simulink model "tractor_mu2018"  (R2018a)
settings: Solver=FixedStepDiscrete  StartTime=0.0  StopTime=30  FixedStep=0.001  RelTol=1e-3
model workspace (MAT data in the model file):
  MCOS : class17 (value not decoded)
undefined symbols (not defined in the file): A, a, B, b, C, D, DiscIntNeverNeededParam, Iz, K, k1, K1, k2, K2, L1, L2, m, magnitude, Phi, Sample_time, Steer_Ratio
libraries: simulink x39, Solver_SF x1, dsparch4 x1
(part 4 of 5)

== matlab function tractor_mu2018/四轮转矩分配/MATLAB Function ==
  data: Mz input; Tfl output; Tfr output; Trl output; Trr output; T0 input; derta input; k input; mode input
function [Tfl,Tfr,Trl,Trr] = fcn(Mz,T0,derta,k,mode)
rf = single(0.834);
rr = single(0.94);
df = single(2.39);
dr = single(2.33);
a = single(2.043);

Trr = single(0);
Trl = single(0);
Tfl = single(0);
Tfr = single(0);


% 强制将输入 Mz 类型设为 single，避免隐式转换
Mz = single(Mz);
T0 = single(T0);
derta = single(derta);
mode = single(mode);

% if mode == 5 || mode == 6
%     k = single(3/7); 
% elseif mode == 1 || mode == 3 
%     k = min(k,1);
%     k = max(k,0.3);
% end

A = T0 / (k + single(1));
B = (Mz - a*sin(derta)*k*A/rf) / (df*cos(derta)*k*rr + dr*rf) * (2*rf*rr);
Trr = (A + B) / single(2);
Trl = (A - B) / single(2);
Tfl = k * Trl;
Tfr = k * Trr;

== matlab function tractor_mu2018/Dugoff轮胎模型/pac2002/rl_dugoff ==
  data: Fz input; Fx0 output; u input; lamda input; alpha input; Fy0 output; Fx output; Fy output
function [Fx0,Fy0,Fx,Fy] = tire(Fz,u,lamda,alpha)
cx = -20;
cy = -20;
L = (1-lamda)/(2*sqrt(cx^2*lamda^2+cy^2*(tan(alpha))^2));
if L<1
    fL = L*(2-L);
else
    fL = 1;
end
Fx0 = Fz*cx*lamda*fL/(1-lamda);
Fy0 = Fz*cy*tan(alpha)*fL/(1-lamda);
Fx = u*Fx0;
Fy = u*Fy0;

== matlab function tractor_mu2018/Dugoff轮胎模型/pac2002/rr_dugoff ==
  data: Fz input; Fx0 output; u input; lamda input; alpha input; Fy0 output; Fx output; Fy output
function [Fx0,Fy0,Fx,Fy] = tire(Fz,u,lamda,alpha)
cx = -20;
cy = -20;
L = (1-lamda)/(2*sqrt((cx^2)*(lamda^2)+(cy^2)*((tan(alpha))^2)));
if L<1
    fL = L*(2-L);
else
    fL = 1;
end
Fx0 = Fz*cx*lamda*fL/(1-lamda);
Fy0 = Fz*cy*tan(alpha)*fL/(1-lamda);
Fx = u*Fx0;
Fy = u*Fy0;

== matlab function tractor_mu2018/质心侧偏角估计/define_Kalman ==
  data: u input; A output; B output; C output; D output; a11 output; a12 output; a21 output single; a22 output; c11 output; c12 output
function [A, B, C, D,a11,a12,a21,a22,c11,c12] = fcn(u)
m = 18530;%质量
Iz = 67536;%绕Z轴的转动惯量
a = 2.043;%前轴距
b=1.362;%后轴距
% k1 = -1360400;%前侧偏刚度
% k2 = -1611200;%后侧偏刚度
k1 = -304828*2;%前侧偏刚度
k2 = -417040*2;%后侧偏刚度
t = 0.001;%仿真步长
Sample_time = 0.001;


a11 = (k1+k2)*t/(m*u)+1;
a12 = ((a*k1-b*k2)/(m*u^2)-1)*t;
a21 = single((a*k1-b*k2)*t/Iz);
a22 = (a^2*k1+b^2*k2)*t/(Iz*u)+1;
b11  =-k1*t/(m*u);
b21 = -a*k1*t/Iz;
c11 = (k1+k2)/m;
c12 = (a*k1-b*k2)/(m*u);
c21 = 0;
c22 = 1;
d11 = -k1/m;
d21 = 0;

%% A B C D 为kalman滤波器中各个矩阵

A = [a11 a12;a21 a22];
B = [b11;b21];
C = [c11 c12;c21 c22];
D = [d11;d21];

== matlab function tractor_mu2018/驱动防滑模块/MATLAB Function ==
  data: sp1 input; vfl output; sp2 input; vfr output
function [vfl,vfr] = fcn(sp1,sp2)
r1 = 0.834;

if sp1>=0
    vfl = max(0.001,sp1*2*pi*r1/60); %m/s
else
    vfl = min(-0.001,sp1*2*pi*r1/60); %m/s
end

if sp2 >= 0
    vfr = max(0.001,sp2*2*pi*r1/60);
else
    vfr = min(0.001,sp2*2*pi*r1/60);
end

== matlab function tractor_mu2018/驱动防滑模块/MATLAB Function1 ==
  data: sp3 input; vrl output; sp4 input; vrr output
function [vrl,vrr] = fcn(sp3,sp4)
r2 = 0.94;

if sp3 >= 0
    vrl = max(0.001,sp3*2*pi*r2/60);
else
    vrl = min(0.001,sp3*2*pi*r2/60);
end

if sp4 >=0
    vrr = max(0.001,sp4*2*pi*r2/60);
else
    vrr = min(0.001,sp4*2*pi*r2/60);
end

== stateflow chart tractor_mu2018/驱动防滑模块/转矩协调控制 ==
  state coordinate
    (default) -> (junction 7)
    (junction 7) -> (junction 9) [order 1] : [dT1 ~= 0]
    (junction 9) -> (junction 11) [order 1] : [dT2 ~= 0]
    (junction 11) -> (junction 14) [order 1] : [abs(dT1)>=abs(dT2)]{dTfr=dT1;dTfl=dT1;}
    (junction 14) -> (junction 16)
    (junction 7) -> (junction 21) [order 2] : {dTfr=dT2;
        | dTfl=dT2}
    (junction 9) -> (junction 19) [order 2] : {dTfr=dT1;
        | dTfl=dT1;}
    (junction 11) -> (junction 16) [order 2] : {dTfr=dT2;dTfl=dT2;}
    (junction 19) -> (junction 21)
    (junction 16) -> (junction 19)
    (junction 21) -> (junction 111)
    (junction 111) -> (junction 106) [order 2] : {dTrr=dT4;
        | dTrl=dT4}
    (junction 111) -> (junction 118) [order 1] : [dT3 ~= 0]
    (junction 118) -> (junction 107) [order 1] : [dT4 ~= 0]
    (junction 107) -> (junction 110) [order 1] : [abs(dT3)>=abs(dT4)]{dTrr=dT3;dTrl=dT3;}
    (junction 110) -> (junction 114)
    (junction 115) -> (junction 106)
    (junction 118) -> (junction 115) [order 2] : {dTrr=dT3;
        | dTrl=dT3;}
    (junction 107) -> (junction 114) [order 2] : {dTrr=dT4;dTrl=dT4;}
    (junction 114) -> (junction 115)
  state no_coordinate
    du:
    dTfl=dT1;
    dTfr=dT2;
    dTrl=dT3;
    dTrr=dT4;
  (default) -> (junction 123)
  (junction 123) -> (junction 126) [order 2]
  (junction 123) -> no_coordinate [order 1] : [v<10]
  (junction 126) -> coordinate
  no_coordinate -> coordinate : [v>=10]
  coordinate -> no_coordinate [order 1] : [v<10]
  coordinate -> coordinate [order 2] : [v>=10]
  data: v input; dT1 input; dT2 input; dT3 input; dT4 input; dTfl output; dTfr output; dTrl output; dTrr output

== matlab function tractor_mu2018/四轮转矩分配/MATLAB Function1 ==
  data: X_current input; U_optimal output; Fx input; Mz input; Fz_all input; mu input; last_U_in input
function U_optimal = mpc_torque_allocation_fcn(X_current, Fx, Mz, Fz_all, mu, last_U_in)
% 基于MPC的四轮驱动车辆扭矩分配。
% 本函数在每个计算步中构建并求解一个二次规划(QP)问题。

%#codegen

% -------------------------------------------------------------------------
% 1. 定义持久化变量和参数
% -------------------------------------------------------------------------
% persistent 关键字定义的变量只在第一次调用函数时初始化，之后会保持它们的值。
persistent vehicle_params mpc_params last_U

if isempty(vehicle_params)
    % --- 车辆参数 ---
    % !! 请根据您的拖拉机模型修改以下参数 !!
    vehicle_params.m = 18530;   % 质量 (kg)
    vehicle_params.Iz = 67536;  % 绕Z轴的转动惯量 (kg*m^2)
    vehicle_params.lf = 2.043;   % 质心到前轴的距离 (m)
    vehicle_params.lr = 1.362;   % 质心到后轴的距离 (m)
    vehicle_params.wf = 2.39;    % 前轮距 (m)
    vehicle_params.wr = 2.33;    % 后轮距 (m)

    % --- MPC 参数 ---
    mpc_params.Ts = 0.001;      % 采样时间 (s)，必须与Simulink的采样时间一致
    mpc_params.Np = 20;        % 预测时域 (Prediction Horizon)
    mpc_params.Nc = 10;         % 控制时域 (Control Horizon)
    
    % --- MPC 权重 ---
    % 对控制输入变化率 (delta U) 的惩罚矩阵R的对角线元素
    mpc_params.R_diag = ones(8, 1) * 0.01; 
    mpc_params.w_ax = 1.0;      % 纵向加速度权重
    mpc_params.w_ay = 1;      % 横向加速度权重
    
    % --- 轮胎附着多边形 ---
    % 使用一个八边形来线性化近似摩擦圆约束
    num_sides = 8;
    angles = (0:num_sides-1)' * (2*pi/num_sides);
    mpc_params.friction_polygon = [cos(angles), sin(angles)]; % [cos, sin] 列
    
    % 初始化上一次的控制输入
    last_U = zeros(8, 1);
end

% 从输入端口更新last_U，以保证时间步之间的一致性
if any(size(last_U_in) ~= size(last_U))
   last_U = zeros(8,1); % 如果是第一次运行或尺寸不匹配，则进行初始化
else
   last_U = last_U_in;
end


% -------------------------------------------------------------------------
% 2. 获取参数
% -------------------------------------------------------------------------
% 车辆参数
m = vehicle_params.m;
Iz = vehicle_params.Iz;
lf = vehicle_params.lf;
lr = vehicle_params.lr;
wf = vehicle_params.wf;
wr = vehicle_params.wr;
bf = wf / 2; % 半轮距
br = wr / 2;

% MPC参数
Ts = mpc_params.Ts;
Np = mpc_params.Np;
Nc = mpc_params.Nc;
R = diag(mpc_params.R_diag);

% 解析输入信号
u_k = X_current(1); % 当前的纵向车速 (m/s)
v_k = X_current(2); % 当前的横向车速 (m/s)
r_k = X_current(3); % 当前横摆角速度 (rad/s)

% -------------------------------------------------------------------------
% 3. 定义状态空间矩阵 
% -------------------------------------------------------------------------
% 连续时间的状态矩阵 A_c，它依赖于当前车速 u_k
A_c = [0, 0, 0;
       0, 0, u_k;
       0, 0, 0];

% 连续时间的输入矩阵 B_c  横摆方向逆时针为正;横向向左为正
B_c = [1/m,   0,   1/m,   0,   1/m,   0,   1/m,   0;
       0,   1/m,   0,   1/m,   0,   1/m,   0,   1/m;
       -bf/Iz, lf/Iz, bf/Iz, lf/Iz, -br/Iz, -lr/Iz, br/Iz, -lr/Iz];

% 使用前向欧拉法进行离散化
Ad = eye(3) + A_c * Ts;
Bd = B_c * Ts;

% -------------------------------------------------------------------------
% 4. 构建二次规划(QP)问题 
%    目标: min 0.5 * dU' * H * dU + f' * dU
% -------------------------------------------------------------------------
% 新代价函数: J = sum( (ax^2+ay^2) + dU'*R*dU )

% ---- 4.1 定义权重和矩阵 ----
% 从参数区获取加速度权重
w_ax = mpc_params.w_ax;
w_ay = mpc_params.w_ay;
Q_accel = diag([w_ax^2, w_ay^2]); % 单步的加速度权重矩阵

% 构建整个控制时域的权重矩阵
Q_bar = kron(eye(Nc), Q_accel);  % 加速度项的权重矩阵
R_bar = kron(eye(Nc), R);      % 控制增量项的权重矩阵

% ---- 4.2 将加速度表示为dU的函数 ----
% 定义一个矩阵，从控制向量U中提取与加速度相关的力
C_u = [1/m, 0, 1/m, 0, 1/m, 0, 1/m, 0;
       0, 1/m, 0, 1/m, 0, 1/m, 0, 1/m];
C_u_bar = kron(eye(Nc), C_u);

% 计算由当前状态(u_k, v_k, r_k)引起的加速度偏移量
% (在线性化过程中被视为常数)
d_accel_k = [-v_k * r_k; 2 * u_k * r_k];
d_accel_bar = repmat(d_accel_k, Nc, 1);

% ---- 4.3 构建QP矩阵 H 和 f ----
% 回忆: U_vec = M_sum * dU_vec + U_last_vec
% 预测的加速度 Accel_vec = C_u_bar * U_vec + d_accel_bar
%                        = C_u_bar * (M_sum * dU_vec + U_last_vec) + d_accel_bar
%                        = (C_u_bar * M_sum) * dU_vec + (C_u_bar * U_last_vec + d_accel_bar)
%
% 令 S = C_u_bar * M_sum
% 令 E = C_u_bar * U_last_vec + d_accel_bar
% 则 Accel_vec = S * dU_vec + E
%
% 加速度部分的代价 J_accel = (S*dU+E)' * Q_bar * (S*dU+E)
% 展开后与QP标准型对比，可以推导出H和f的构成

% 预先计算一个将 dU_vec 映射到 U_vec 的矩阵
% U_vec = M_sum * dU_vec + U_last_vec
M_sum = kron(tril(ones(Nc, Nc)), eye(8));
U_last_vec = repmat(last_U, Nc, 1);

S = C_u_bar * M_sum;
E = C_u_bar * U_last_vec + d_accel_bar;

% 构建 H 矩阵
H = 2 * (S' * Q_bar * S + R_bar);

% 构建 f 向量
f = 2 * (S' * Q_bar * E);

% ---- 4.2 构建约束矩阵 ----
% 优化变量是dU。所有约束都必须是关于dU的线性形式: A*dU <= b 或 Aeq*dU = beq
% 未来的控制量 U_k+i 与 增量 dU 的关系: U_k+i = U_{k-1} + dU_k + ... + dU_k+i



% --- 4.2.1 等式约束: Aeq * dU_vec = beq ---
% 在所有 Nc 控制步内，都满足 Fx_total = Fx_ref 和 Mz_total = Mz_ref
C_fx = [1, 0, 1, 0, 1, 0, 1, 0];
C_mz = [-bf, lf, bf, lf, -br, -lr, br, -lr]; % 注意: 此处未除以Iz，因为约束是针对力矩本身

Aeq_block = [C_fx; C_mz]; % (维度: 2 x 8)
Aeq = kron(eye(Nc), Aeq_block); % (维度: 2*Nc x 8*Nc)
Aeq = Aeq * M_sum;

% 构建等式约束右侧的beq向量
beq_fx = ones(Nc, 1) * Fx;
beq_mz = ones(Nc, 1) * Mz;
beq_block = [beq_fx'; beq_mz']; % (维度: 2 x Nc)
beq = beq_block(:); % (维度: 2*Nc x 1)
% 别忘了减去上个时刻控制量的影响
beq = beq - kron(eye(Nc), Aeq_block) * U_last_vec;

% --- 4.2.2 不等式约束: Aineq * dU_vec <= bineq ---
% 对所有4个轮胎、在所有Nc控制步内的轮胎附着多边形约束
% poly_sides = mpc_params.friction_polygon;
% num_sides = size(poly_sides, 1);
% num_tires = 4;
% 
% Aineq_block = zeros(num_sides * num_tires, 8);
% for i = 1:num_tires % 遍历: 左前, 右前, 左后, 右后
%     % 找到这个轮胎对应的Fx和Fy列的索引
%     idx_fx = 2*i - 1;
%     idx_fy = 2*i;
%     
%     % 获取这个轮胎对应约束的行索引范围
%     row_start = (i-1)*num_sides + 1;
%     row_end = i*num_sides;
%     
%     % 填充多边形约束系数
%     Aineq_block(row_start:row_end, idx_fx) = poly_sides(:, 1); % cos(theta)
%     Aineq_block(row_start:row_end, idx_fy) = poly_sides(:, 2); % sin(theta)
% end
% 
% Aineq = kron(eye(Nc), Aineq_block); % (维度: num_sides*num_tires*Nc x 8*Nc)
% Aineq = Aineq * M_sum;
% 
% % 构建不等式约束右侧的bineq向量
% mu_vec = ones(4,1) * mu; % 暂时假设所有轮胎的附着系数 mu 相同
% Fz_mu_vec = Fz_all .* mu_vec; % 计算每个轮胎的最大附着力
% bineq_block = repelem(Fz_mu_vec, num_sides, 1); % repelem for R2017a+, for older use kron
% bineq = repmat(bineq_block, Nc, 1);
% % 同样，减去上个时刻控制量的影响
% bineq = bineq - kron(eye(Nc), Aineq_block) * U_last_vec;

% -------------------------------------------------------------------------
% 5. 求解QP问题
% -------------------------------------------------------------------------
% 设置 quadprog 求解器选项
U_optimal = zeros(8,1);
options = optimoptions('quadprog', 'Display', 'none', 'Algorithm', 'active-set');

% 为求解器创建一个全零的初始猜测点 x0
% 它的维度必须与优化变量dU_vec一致 (8*Nc x 1)
x0 = zeros(8 * Nc, 1);

% --- 【新增代码】构建下界(lb)向量以保证驱动轮Fx >= 0 ---
% lb是直接作用于优化变量dU_vec的

% 首先，为单个时间步的dU创建一个下界向量
lb_step = -inf(8, 1);

% 假设所有4个轮子都只作为驱动轮，不能为负
% Fx的索引是 1, 3, 5, 7
drive_idx = [1, 3, 5, 7]; 
% Fx的增量的下界是上一时刻Fx的负值，以保证 Fx_k = Fx_{k-1} + dFx_k >= 0
lb_step(drive_idx) = -last_U(drive_idx);

% 然后，将单步的下界向量复制Nc次，以覆盖整个控制时域
lb = repmat(lb_step, Nc, 1);

% 【修改代码】调用求解器，将lb作为第7个参数传入
% [dU_vec_sol, ~, exitflag] = quadprog(H, f, Aineq, bineq, Aeq, beq, lb, [], x0, options);
[dU_vec_sol, ~, exitflag] = quadprog(H, f, [], [], Aeq, beq, lb, [], x0, options);
% -------------------------------------------------------------------------
% 6. 处理求解结果
% -------------------------------------------------------------------------
if exitflag == 1 % 返回1代表求解成功
    % 提取第一个控制增量 (Receding Horizon Control)
    dU_optimal = dU_vec_sol(1:8);
    % 计算当前时刻的最终控制输入
    U_optimal = last_U + dU_optimal;
else
    % 如果求解失败, 保持上一次的控制输入不变 (作为一种安全备用策略)
    U_optimal = last_U;
end

% 无需在此更新 last_U, 因为它会作为输出连接到Unit Delay模块，
% 并在下个采样时刻通过输入端口 last_U_in 传回。

end

== matlab function tractor_mu2018/Subsystem/MATLAB Function ==
  data: Fd input; P_qianyin input; y output; P_qudong input; v input
function y = fcn(Fd,P_qianyin,P_qudong,v)

if Fd > 0 && v > 0.5/3.6
    y = P_qianyin/P_qudong;
else
    y = 0;
end
if P_qudong < 2000
    y = 0;
end

== matlab function tractor_mu2018/四轮转矩分配/MATLAB Function2 ==
  data: F input; Tfl output; derta input; Tfr output; Trl output; Trr output; dwfl input; dwfr input; dwrl input; dwrr input
function [Tfl,Tfr,Trl,Trr] = fcn(F,derta,dwfl,dwfr,dwrl,dwrr)
% 向左为正
rf = 0.834;
rr = 0.94;
If = 110.64; % kg*m^2
Ir = 356.42;

Ffl = F(1)*cos(derta) + F(2)*sin(derta);
Tfl = Ffl*rf + If*dwfl;
Ffr = F(3)*cos(derta) + F(4)*sin(derta);
Tfr = Ffr*rf + If*dwfr;
Frl = F(5);
Trl = Frl*rr + Ir*dwrl;
Frr = F(7);
Trr = Frr*rr + Ir*dwrr;

== matlab function tractor_mu2018/驱动防滑模块/MATLAB Function2 ==
  data: v input; dTfl output; dT1 input; dT2 input; dT3 input; dT4 input; dTfr output; dTrl output; dTrr output
function [dTfl,dTfr,dTrl,dTrr] = fcn(v,dT1,dT2,dT3,dT4)

v = v*3.6;

if v < 1.5
    dTfl = 0;
    dTfr = 0;
    dTrl = 0;
    dTrr = 0;
end

if v < 10
    dTfl = dT1;
    dTfr = dT2;
    dTrl = dT3;
    dTrr = dT4;
else 
    if abs(dT1) > abs(dT2)
        dTfl = dT1;
        dTfr = dT1;
    else
        dTfl = dT2;
        dTfr = dT2;
    end
    if abs(dT3) > abs(dT4)
        dTrl = dT3;
        dTrr = dT3;
    else
        dTrl = dT4;
        dTrr = dT4;
    end
end

== stateflow chart tractor_mu2018/车轮腾空判断/FL ==
  state suspected
    airborne_flag = 0; confidence = 0.5;
  state grounded
    airborne_flag = 0; confidence = 0;
  state airborne
    airborne_flag = 1; confidence = 1;
  grounded -> suspected : [ (lamda > 0) && (Tload_hat < 50) && (domega > 0) && (abs(az)) > 2]
  suspected -> airborne : [after(0.02, sec)]
  (default) -> grounded
  airborne -> grounded : [(lamda < 0.02) && (Tload_hat > 100) && abs(az) < 1 && after(0.05,sec)]
  data: lamda input; Tload_hat input; az input; domega input; airborne_flag output; confidence output

== stateflow chart tractor_mu2018/车轮腾空判断/FR ==
  state suspected
    airborne_flag = 0; confidence = 0.5;
  state grounded
    airborne_flag = 0; confidence = 0;
  state airborne
    airborne_flag = 1; confidence = 1;
  grounded -> suspected : [ (lamda > 0) && (Tload_hat < 50) && (domega > 0) && (abs(az)) > 2]
  suspected -> airborne : [after(0.02, sec)]
  (default) -> grounded
  airborne -> grounded : [(lamda < 0.02) && (Tload_hat > 100) && abs(az) < 1 && after(0.05,sec)]
  data: lamda input; Tload_hat input; az input; domega input; airborne_flag output; confidence output

== stateflow chart tractor_mu2018/车轮腾空判断/RL ==
  state suspected
    airborne_flag = 0; confidence = 0.5;
  state grounded
    airborne_flag = 0; confidence = 0;
  state airborne
    airborne_flag = 1; confidence = 1;
  grounded -> suspected : [ (lamda > 0) && (Tload_hat < 50) && (domega > 0) && (abs(az)) > 2]
  suspected -> airborne : [after(0.02, sec)]
  (default) -> grounded
  airborne -> grounded : [(lamda < 0.02) && (Tload_hat > 100) && abs(az) < 1 && after(0.05,sec)]
  data: lamda input; Tload_hat input; az input; domega input; airborne_flag output; confidence output

== stateflow chart tractor_mu2018/车轮腾空判断/RR ==
  state suspected
    airborne_flag = 0; confidence = 0.5;
  state grounded
    airborne_flag = 0; confidence = 0;
  state airborne
    airborne_flag = 1; confidence = 1;
  grounded -> suspected : [ (lamda > 0) && (Tload_hat < 50) && (domega > 0) && (abs(az)) > 2]
  suspected -> airborne : [after(0.02, sec)]
  (default) -> grounded
  airborne -> grounded : [(lamda < 0.02) && (Tload_hat > 100) && abs(az) < 1 && after(0.05,sec)]
  data: lamda input; Tload_hat input; az input; domega input; airborne_flag output; confidence output

== matlab function tractor_mu2018/驱动防滑模块/MATLAB Function3 ==
  data: vfl input; v output; vfr input; vrl input; vrr input; omega input; brk input; st input
function v = fcn(vfl,vfr,vrl,vrr,omega,brk,st)
d = 2.36;
brk_bank = 40;
st_bank = 10;

v = 0;
if abs(st) <= st_bank && brk < brk_bank
    v = min([vfl,vfr,vrl,vrr]);
elseif abs(st) <= st_bank && brk >= brk_bank
    v = max([vfl,vfr,vrl,vrr]);
elseif abs(st) > st_bank && brk >= brk_bank
    v = 0.5*max([vfl+vrl-d*omega,vfr+vrr+d*omega]);
elseif abs(st) > st_bank && brk < brk_bank
    v = 0.5*max([vfl+vrl-d*omega,vfr+vrr+d*omega]);
end

== matlab function tractor_mu2018/质心侧偏角滑模观测器估计/Subsystem/MATLAB Function ==
  data: vx input; d_vy_model output; delta_f input; vy_hat input; gamma_hat input; d_gamma_model output
function [d_vy_model, d_gamma_model] = fcn(vx, delta_f, vy_hat, gamma_hat)

% 声明我们将使用来自MATLAB基础工作区的参数
m = 18530;%质量
Iz = 67536;%绕Z轴的转动惯量
a = 2.043;%前轴距
b=1.362;%后轴距
% Cf = 1360400;%前侧偏刚度
% Cr = 1611200;%后侧偏刚度
 Cf = 304828*2;Cr = 417040*2; % 仿真用

% 防止vx为0导致计算错误
if abs(vx) < 0.1
    vx = 0.1;
end

% 二自由度模型方程
d_vy_model = (-(Cf + Cr) / (m * vx)) * vy_hat + ...
             ((b * Cr - a * Cf) / (m * vx) - vx) * gamma_hat + ...
             (Cf / m) * delta_f;

d_gamma_model = ((b * Cr - a * Cf) / (Iz * vx)) * vy_hat - ...
                ((a^2 * Cf + b^2 * Cr) / (Iz * vx)) * gamma_hat + ...
                (a * Cf / Iz) * delta_f;

== matlab function tractor_mu2018/质心侧偏角滑模观测器估计/Subsystem1/MATLAB Function ==
  data: vx input; d_vy_model output; delta_f input; vy_hat input; gamma_hat input; d_gamma_model output
function [d_vy_model, d_gamma_model] = fcn(vx, delta_f, vy_hat, gamma_hat)

% 声明我们将使用来自MATLAB基础工作区的参数
m = 18530;%质量
Iz = 67536;%绕Z轴的转动惯量
a = 2.043;%前轴距
b=1.362;%后轴距
Cf = 1360400;%前侧偏刚度
Cr = 1611200;%后侧偏刚度

% 防止vx为0导致计算错误
if abs(vx) < 0.1
    vx = 0.1;
end

% 二自由度模型方程
d_vy_model = (-(Cf + Cr) / (m * vx)) * vy_hat + ...
             ((b * Cr - a * Cf) / (m * vx) - vx) * gamma_hat + ...
             (Cf / m) * delta_f;

d_gamma_model = ((b * Cr - a * Cf) / (Iz * vx)) * vy_hat - ...
                ((a^2 * Cf + b^2 * Cr) / (Iz * vx)) * gamma_hat + ...
                (a * Cf / Iz) * delta_f;

== matlab function tractor_mu2018/PF车速估计 ==
  data: ax_m input; vx_est output; ay_m input; r_m input; vy_est output; init_vx input; init_vy input
function [vx_est, vy_est] = fcn_ImprovedPF(ax_m, ay_m, r_m, init_vx, init_vy)
% 基于改进粒子滤波的车速估计
% 严格按照论文公式 (5)-(19) 实现

% --- 参数定义 (可根据实际情况调整) ---
persistent particles weights first_run
persistent T mx my mr Q R

if isempty(first_run)
    % 初始化参数
    N = 200; % 粒子数量 (论文伪代码步骤 0)
    T = 0.01; % 采样时间，对应传感器更新频率 (0.01s)
    
    % 自定义常数 (公式 17) - 需要根据调试确定
    mx = 0.5; 
    my = 0.5;
    mr = 0.1;
    
    % 过程噪声标准差 (公式 12 & 18) - 这里的 u 对应 xi
    sigma_proc = [0.1; 0.1; 0.01]; % [xi_x, xi_y, xi_z]
    Q = diag(sigma_proc.^2); 

    % 观测噪声标准差 (公式 13)
    sigma_meas = [0.2; 0.2; 0.01]; % [omega_ax, omega_ay, omega_r]
    R = diag(sigma_meas.^2);
    
    % --- 1. 初始化滤波器 (论文伪代码步骤 1) ---
    % 状态向量 X = [vx, ax, vy, ay, r]' (5维)
    % 粒子初始化：在初始值附近添加随机扰动
    particles = zeros(5, N);
    particles(1, :) = init_vx + randn(1, N) * 0.5; % vx
    particles(2, :) = ax_m + randn(1, N) * 0.1;    % ax
    particles(3, :) = init_vy + randn(1, N) * 0.1; % vy
    particles(4, :) = ay_m + randn(1, N) * 0.1;    % ay
    particles(5, :) = r_m + randn(1, N) * 0.01;    % r
    
    weights = ones(1, N) / N; % 初始化权重
    
    first_run = 0;
end

N = size(particles, 2);
particles_next = zeros(5, N);

% 测量向量 Z_k (公式 13上方定义)
Z_k = [ax_m; ay_m; r_m]; 

% --- 2. 粒子滤波主循环 ---
% 对应论文伪代码的步骤 2-8 (针对每个时刻)

% 预计算 G 矩阵的一部分 (公式 11) 和 L 矩阵的一部分 (公式 17)
% 注意：G 和 L 实际上在每个粒子计算中略有不同吗？
% 论文中 G 是常数矩阵，但 L 取决于测量值与上一时刻状态的差，
% 且公式 (19) X_k = F*X_k-1 + P_k + G*L*xi
% 这里我们需要对每个粒子进行循环

for i = 1:N
    % 提取第 i 个粒子上一时刻的状态 X_k-1
    X_prev = particles(:, i);
    vx_prev = X_prev(1);
    ax_prev = X_prev(2);
    vy_prev = X_prev(3);
    ay_prev = X_prev(4);
    r_prev  = X_prev(5);
    
    % --- 计算状态转移矩阵 F_k (公式 10) ---
    % 注意：原论文公式(10)中有笔误，第二行和第四行应该是全0行还是保持加速度不变？
    % 通常 CA (Constant Acceleration) 模型加速度导数为0。
    % 论文公式(10) F_k 矩阵：
    % Row 1: vx = vx + ax*T + vy*r*T (源自 ax = vx_dot - vy*r -> vx_dot = ax + vy*r) -> 离散化: vx_k = vx_k-1 + ax_k-1*T + vy_k-1*r_k-1*T (对应公式 7)
    % Row 2: ax = ax (常数模型) -> 0 1 0 0 0
    % Row 3: vy = vy + ay*T - vx*r*T (源自 ay = vy_dot + vx*r -> vy_dot = ay - vx*r) -> 离散化: vy_k = vy_k-1 + ay_k-1*T - vx_k-1*r_k-1*T (对应公式 8)
    % Row 4: ay = ay -> 0 0 0 1 0
    % Row 5: r = r -> 0 0 0 0 1
    
    F_k = [1, T,  r_prev*T, 0, 0;
           0, 1,         0, 0, 0;
          -r_prev*T, 0,  1, T, 0;
           0, 0,         0, 1, 0;
           0, 0,         0, 0, 1];
       
    % --- 3. 计算提议分布修正项 P_k (公式 14) ---
    % 论文中 a_x,k-1 是粒子状态，而 Z 中的 a_x 是当前测量值。
    % 公式 (14) 利用了测量值与粒子状态的差值。
    % 注意下标：公式里用的是 k-1 时刻的测量值和粒子，但在实时运行中，我们通常拿当前测量值去修正预测。
    % 也就是论文提到的 "基于 k-1 时刻传感器测量值...与 k-1 时刻每个粒子的...差值"。
    % 这里为了代码简洁，假设输入的 ax_m 即为 k-1 时刻（或者当前时刻用来修正前一步）。
    % 严格照公式：
    diff_ax = ax_m - ax_prev; % (a_xz,k-1 - a^i_x,k-1)
    diff_ay = ay_m - ay_prev; % (a_yz,k-1 - a^i_y,k-1)
    diff_r  = r_m  - r_prev;  % (r_z,k-1 - r^i_k-1)
    
    P_k = [T * (diff_ax + diff_r); % 第一行对应 vx 的修正
           diff_ax;                % 第二行对应 ax 的修正
           T * (diff_ay + diff_r); % 第三行对应 vy 的修正
           diff_ay;                % 第四行对应 ay 的修正
           diff_r];                % 第五行对应 r  的修正
           
    % --- 计算自适应增益矩阵 L_k (公式 17) ---
    L_k = [mx * diff_ax, 0, 0;
           0, my * diff_ay, 0;
           0, 0, mr * diff_r];
       
    % --- 计算过程噪声矩阵 G (公式 11) ---
    G = [T^2/2, 0, 0;
         T,     0, 0;
         0, T^2/2, 0;
         0, T,     0;
         0, 0,     T];
         
    % --- 生成标准高斯噪声 xi (公式 18) ---
    % xi 对应伪代码中的 "相互独立的标准高斯噪声"
    xi = randn(3, 1); 
    
    % --- 4. 状态预测 (公式 19) ---
    % X_k = F_k * X_k-1 + P_k + G * L_k * xi
    particles_next(:, i) = F_k * X_prev + P_k + G * L_k * xi;
    
    % --- 5. 权重更新 (伪代码步骤 6 & 7) ---
    % 计算该粒子的预测观测值 Z_pre (公式 13)
    % Z = [ax, ay, r]'
    % 状态向量 X = [vx, ax, vy, ay, r]' -> 对应的索引是 2, 4, 5
    Z_pre = [particles_next(2, i); 
             particles_next(4, i); 
             particles_next(5, i)];
         
    % 计算似然 (高斯分布)
    % likelihood = (1/sqrt((2*pi)^3 * det(R))) * exp(-0.5 * (Z_k - Z_pre)' * inv(R) * (Z_k - Z_pre));
    % 简化计算 (忽略常数项，因为最后会归一化)
    error = Z_k - Z_pre;
    likelihood = exp(-0.5 * (error' / R * error));
    
    weights(i) = weights(i) * likelihood;
end

% --- 6. 权重归一化 (伪代码步骤 10) ---
sum_weights = sum(weights);
if sum_weights > 0
    weights = weights / sum_weights;
else
    weights = ones(1, N) / N; % 防止除以零
end

% --- 7. 重采样 (伪代码步骤 9) ---
% 有效粒子数 (N_eff) 判断是否需要重采样
N_eff = 1 / sum(weights.^2);
if N_eff < N / 2
    particles_next = Resample(particles_next, weights, N);
    weights = ones(1, N) / N;
end

% 更新粒子集
particles = particles_next;

% --- 8. 输出状态估计 (伪代码步骤 11) ---
% 加权平均
vx_est = sum(particles(1, :) .* weights);
vy_est = sum(particles(3, :) .* weights);

end

% --- 辅助函数：重采样 (Systematic Resampling) ---
function new_particles = Resample(particles, weights, N)
    cdf = cumsum(weights);
    new_particles = zeros(size(particles));
    u = rand / N;
    j = 1;
    for i = 1:N
        u_i = u + (i - 1) / N;
        while u_i > cdf(j)
            j = j + 1;
            if j > N, j = N; end
        end
        new_particles(:, i) = particles(:, j);
    end
end

== matlab function tractor_mu2018/加速度滑模观测/MATLAB Function ==
  data: gamma_m input; phi_est output; phi_GPS input; GPS_valid input; gamma_corrected output; e_gamma_est output
function [phi_est, gamma_corrected, e_gamma_est] = GPS_INS_SlidingMode(gamma_m, phi_GPS, GPS_valid)
%% GPS/INS融合 - 滑模观测器
% 输入:
%   gamma_m   - INS测量的横摆角速度 (rad/s)
%   phi_GPS   - GPS测量的航向角 (rad)
%   GPS_valid - GPS数据有效标志
% 输出:
%   phi_est         - 估计的航向角 (rad)
%   gamma_corrected - 校正后的横摆角速度 (rad/s)
%   e_gamma_est     - 估计的横摆角速度偏差 (rad/s)

%% 参数设置
persistent phi_hat e_gamma_hat phi_GPS_last initialized

dt_sim = 0.001;      % 仿真步长 (s)

% ===== 滑模增益（主要调参对象）=====
k1 = 5;              % 航向角校正增益
k2 = 0.5;            % 角速度偏差校正增益
lambda = 10;         % 滑模面斜率

% 边界层厚度（消除抖振）
epsilon = 0.01;      % 越小越精确，但抖振越大

%% 初始化
if isempty(initialized)
    phi_hat = 0;
    e_gamma_hat = 0;
    phi_GPS_last = 0;
    initialized = true;
end

%% 滑模观测器核心算法

% 状态方程：
% phi_dot = gamma_m - e_gamma（真实角速度 = 测量值 - 偏差）
% e_gamma_dot ≈ 0（偏差缓慢变化）

if GPS_valid
    % 滑模面：s = phi_GPS - phi_hat
    s = phi_GPS - phi_hat;
    
    % 饱和函数（替代sign函数，减少抖振）
    if abs(s) > epsilon
        sat_s = sign(s);
    else
        sat_s = s / epsilon;
    end
    
    % 滑模观测器方程
    % 航向角估计
    phi_hat_dot = (gamma_m - e_gamma_hat) + k1 * sat_s;
    
    % 角速度偏差估计（利用滑模的等效控制）
    e_gamma_hat_dot = -k2 * sat_s;
    
    % 积分更新
    phi_hat = phi_hat + phi_hat_dot * dt_sim;
    e_gamma_hat = e_gamma_hat + e_gamma_hat_dot * dt_sim;
    
    % 保存GPS值
    phi_GPS_last = phi_GPS;
    
else
    % GPS无效时，纯惯性推算
    phi_hat = phi_hat + (gamma_m - e_gamma_hat) * dt_sim;
    % e_gamma_hat 保持不变
end

%% 输出
phi_est = phi_hat;
e_gamma_est = e_gamma_hat;
gamma_corrected = gamma_m - e_gamma_hat;

end

== matlab function tractor_mu2018/加速度滑模观测/MATLAB Function1 ==
  data: a_xm input; a_xc output; a_ym input; v_xGPS input; v_yGPS input; gamma_c input; GPS_update_flag input; a_yc output; e_ax_est output; e_ay_est output; reset input
function [a_xc, a_yc, e_ax_est, e_ay_est] = accel_SMO_correction(a_xm, a_ym, v_xGPS, v_yGPS, gamma_c, GPS_update_flag, reset)
% 加速度滑模观测器校正
% 输入：
%   a_xm, a_ym      - INS测量的加速度 (m/s^2)
%   v_xGPS, v_yGPS  - GPS测量的速度 (m/s)
%   gamma_c         - 校正后的横摆角速度 (rad/s)
%   GPS_update_flag - GPS更新标志 (1=有新数据)
%   reset           - 复位信号
% 输出：
%   a_xc, a_yc      - 校正后的加速度
%   e_ax_est, e_ay_est - 估计的加速度偏差

% 采样时间
dt = 0.001;     % 仿真步长
DT = 0.05;      % GPS采样周期

% 滑模观测器增益（需根据实际调参）
persistent k1 k2 lambda1 lambda2
if isempty(k1)
    k1 = 5;       % 速度误差增益
    k2 = 5;
    lambda1 = 0.5; % 加速度偏差增益
    lambda2 = 0.5;
end

% 持久变量（状态记忆）
persistent v_xI v_yI e_ax e_ay initialized
persistent a_xm_sum a_ym_sum sum_count

if isempty(initialized) || reset
    v_xI = 0;      % INS积分速度 x
    v_yI = 0;      % INS积分速度 y
    e_ax = 0;      % 加速度偏差估计 x
    e_ay = 0;      % 加速度偏差估计 y
    a_xm_sum = 0;  % 加速度累加（用于GPS周期内求和）
    a_ym_sum = 0;
    sum_count = 0;
    initialized = true;
end

% 累加加速度（对应论文中的求和项）
a_xm_sum = a_xm_sum + a_xm;
a_ym_sum = a_ym_sum + a_ym;
sum_count = sum_count + 1;

% 速度积分（考虑横摆角速度耦合，对应式3-10）
% v_xI(k+1) = v_xI(k) + dt*a_xm + DT*(v_yI*gamma_c - e_ax - n_ax)
% 简化：每步用校正后的加速度积分
a_xc_temp = a_xm - e_ax;
a_yc_temp = a_ym - e_ay;

% 考虑横摆角速度耦合的速度更新
v_xI = v_xI + dt * (a_xc_temp + v_yI * gamma_c);
v_yI = v_yI + dt * (a_yc_temp - v_xI * gamma_c);

% GPS更新时刻：执行滑模校正
if GPS_update_flag == 1
    % 速度误差（观测残差）
    e_vx = v_xI - v_xGPS;
    e_vy = v_yI - v_yGPS;
    
    % 滑模切换函数
    s_x = sign(e_vx);
    s_y = sign(e_vy);
    
    % 也可用饱和函数避免抖振
    % epsilon = 0.1;
    % s_x = sat_func(e_vx, epsilon);
    % s_y = sat_func(e_vy, epsilon);
    
    % 速度校正（直接用GPS速度重置，或软校正）
    % 软校正方式：
    v_xI = v_xI - k1 * DT * s_x;
    v_yI = v_yI - k2 * DT * s_y;
    
    % 加速度偏差更新（滑模观测器核心）
    e_ax = e_ax + lambda1 * DT * s_x;
    e_ay = e_ay + lambda2 * DT * s_y;
    
    % 限幅防止发散
    e_ax = max(min(e_ax, 2), -2);
    e_ay = max(min(e_ay, 2), -2);
    
    % 清零累加器
    a_xm_sum = 0;
    a_ym_sum = 0;
    sum_count = 0;
end

% 输出校正后的加速度（式3-12）
a_xc = a_xm - e_ax;
a_yc = a_ym - e_ay;

% 输出偏差估计（用于调试）
e_ax_est = e_ax;
e_ay_est = e_ay;

end

% 饱和函数（可选，减少抖振）
function y = sat_func(x, epsilon)
    if abs(x) <= epsilon
        y = x / epsilon;
    else
        y = sign(x);
    end
end

== matlab function tractor_mu2018/质心侧偏角观测/MATLAB Function ==
  data: x_hat input; x_dot output; u input; z_meas input; z_hat output
function [x_dot, z_hat] = fcn(x_hat, u, z_meas)

    % === 车辆物理参数 ===
    mv = 18530;       % Vehicle total mass (kg)
    Izz = 67536;      % Second moment of mass (kg m^2)
    L1 = 2.043;        % CG to front axle (m)
    L2 = 1.362;        % CG to rear axle (m)
    Cf1 = 304828 * 2;     % Front cornering stiffness (N/rad) - 对应图中 C_F\delta^1
    Cf2 = 417040 * 2;     % Rear cornering stiffness (N/rad) - 对应图中 C_F\delta^2

    % === 观测器参数===
    Lambda = [100, 0;    % 增益矩阵 (3x2)
          0, 100;    
          0, 1000];   
    lambda_param = 1;
    Ts = 0.001;           % 离散采样时间 (Discrete Sample Time)

    % === 1. 解包状态变量和输入 ===
    % x_hat = [Vg_est; delta_est; r_est] 
    x1 = x_hat(1); % V_G
    x2 = x_hat(2); % delta (侧偏角)
    x3 = x_hat(3); % psi_dot (横摆角速度)

    % u = [beta; Fl1; Fl2]
    u1 = u(1); % beta
    u2 = u(2); % Fl1
    u3 = u(3); % Fl2
    
    % 防止分母为0
    if abs(x1) < 0.1
        x1 = 0.1; 
    end

    % === 2. 计算估计的输出 z_hat  ===
    % z = [Vg; psi_dot]
    h_NL = [x1; x3]; 
    z_hat = h_NL;

    % === 3. 计算观测误差 (z - z_hat) ===
    error = z_meas - z_hat;

    % === 4. 计算 Sign_eq 函数 ===
    sign_term = (2/pi) * atan(lambda_param * error);

    % === 5. 计算非线性函数 ===
    term1_1 = (1/mv) * (u2 * cos(x2 - u1) + u3 * cos(x2));
    term1_2 = (1/mv) * Cf2 * (-x2 + L2*x3/x1) * sin(x2);
    term1_3 = (1/mv) * Cf1 * (u1 - x2 - L1*x3/x1) * sin(x2 - u1);
    
    dx1_val = term1_1 + term1_2 + term1_3;

    term2_1 = 1/(mv*x1) * (u2 * sin(u1 - x2) - u3 * sin(x2)) ;
    term2_2 = 1/(mv*x1) * Cf1 * (u1 - x2 - L1*x3/x1) * cos(u1 - x2);
    term2_3 = 1/(mv*x1) * Cf2 * (-x2 + L2*x3/x1) * cos(x2) - x3;
    
    dx2_val = term2_1 + term2_2 + term2_3;

    term3_1 = (1/Izz) * ( L1 * u2 * sin(u1) - L2 * Cf2 * (-x2 + L2*x3/x1) ); 
    term3_2 = (1/Izz) * L1 * Cf1 * (u1 - x2 - L1*x3/x1) * cos(u1);
    
    dx3_val = term3_1 + term3_2;
    
    f_NL = [dx1_val; dx2_val; dx3_val];

    % === 6. 最终观测器状态导数 ===
    % x_hat_dot = f_NL(x_hat, u) + Lambda * sign_eq(z - z_hat)
    x_dot = f_NL + Lambda * sign_term;
end

== matlab function tractor_mu2018/Subsystem/计算平均边际贡献 ==
  data: v_all input; phi output
function phi = shapley_calc(v_all)

% 输入:
% v_all: 16x1
%
% 子集顺序:
%
% 1  -> []
% 2  -> [1]
% 3  -> [2]
% 4  -> [3]
% 5  -> [4]
% 6  -> [1 2]
% 7  -> [1 3]
% 8  -> [1 4]
% 9  -> [2 3]
% 10 -> [2 4]
% 11 -> [3 4]
% 12 -> [1 2 3]
% 13 -> [1 2 4]
% 14 -> [1 3 4]
% 15 -> [2 3 4]
% 16 -> [1 2 3 4]
%
% 输出:
% phi = [FL; FR; RL; RR]

%% 平移法消除负值

v_min = min(v_all);

if v_min < 0
    v_all = v_all - v_min;
end

%% 参数

n = 4;

fact = factorial(0:n);

phi = zeros(4,1);

%% 联盟定义

coalitions = [...
    0 0 0 0;  % 1
    1 0 0 0;  % 2
    0 1 0 0;  % 3
    0 0 1 0;  % 4
    0 0 0 1;  % 5
    1 1 0 0;  % 6
    1 0 1 0;  % 7
    1 0 0 1;  % 8
    0 1 1 0;  % 9
    0 1 0 1;  % 10
    0 0 1 1;  % 11
    1 1 1 0;  % 12
    1 1 0 1;  % 13
    1 0 1 1;  % 14
    0 1 1 1;  % 15
    1 1 1 1]; % 16

%% Shapley计算

for i = 1:n

    for idx = 1:16

        S = coalitions(idx,:);

        % 若联盟中已有玩家i
        if S(i) == 1
            continue;
        end

        % 联盟大小
        k = sum(S);

        % 权重
        w = fact(k+1) * fact(n-k) / fact(n+1);

        % v(S)
        v_S = v_all(idx);

        % 构造 S∪{i}
        S_with_i = S;
        S_with_i(i) = 1;

        %% 查找 S∪{i} 对应索引

        idx_Si = 1;

        for j = 1:16

            if isequal(coalitions(j,:), S_with_i)

                idx_Si = j;
                break;

            end

        end

        % v(S∪{i})
        v_Si = v_all(idx_Si);

        % Shapley累加
        phi(i) = phi(i) + w * (v_Si - v_S);

    end

end

phi_min = min(phi);

if phi_min < 0
    phi = phi - phi_min;
end

end

== matlab function tractor_mu2018/Subsystem1/MATLAB Function ==
  data: v input; alpha output
function alpha = fcn(v)

if v < 0.5
    alpha = 0;
elseif v < 5
    alpha = (v - 0.5)/(5 - 0.5);
else
    alpha = 1;
end

== matlab function tractor_mu2018/Subsystem/MATLAB Function3 ==
  data: Fx input; V_all output; Vx input; T input; uF input; mu input; Fz input; slip input; Mz_ref input; Traction_all output; lamdaN_all output; lamda_all output; Mz_all output
function [V_all,Traction_all,lamdaN_all,lamda_all,Mz_all] = shapley_value_all(...
Fx,...
Vx,...
T,...
uF,...
mu,...
Fz,...
slip,...
Mz_ref)

%% 参数

kf = 3;   % 前轮牵引权重
kr = 6;   % 后轮牵引权重

w1 = 100000;  % 滑转率损失权重
w2 = 5000;    % 附着利用率均衡权重
w3 = 0.0001;  % 横摆稳定损失权重

% 半轮距
bf = 2.39/2;
br = 2.33/2;

%% 初始化

V_all = zeros(16,1);
Traction_all = zeros(16,1);
lamdaN_all = zeros(16,1);
lamda_all = zeros(16,1);
Mz_all = zeros(16,1);

%% 16个联盟

coalitions = [...
    0 0 0 0;  % 空集-1
    1 0 0 0;  % 2
    0 1 0 0;  % 3
    0 0 1 0;  % 4
    0 0 0 1;  % 5
    1 1 0 0;  % 6
    1 0 1 0;  % 7
    1 0 0 1;  % 8
    0 1 1 0;  % 9
    0 1 0 1;  % 10
    0 0 1 1;  % 11
    1 1 1 0;  % 12
    1 1 0 1;  % 13
    1 0 1 1;  % 14
    0 1 1 1;  % 15
    1 1 1 1];  % 16

%% 遍历所有联盟

for k = 1:16

    coalition = coalitions(k,:)';

    %% 联盟数据

    Fx_s    = Fx    .* coalition;
    T_s     = T     .* coalition;
    uF_s    = uF   .* coalition;
    mu_s    = mu    .* coalition;
    Fz_s    = Fz    .* coalition;
    slip_s  = slip   .* coalition;

    %% 1 牵引能力项

    F_front = uF_s(1) + uF_s(2);
    F_rear  = uF_s(3) + uF_s(4);

    traction_term = ...
        kf * F_front + ...
        kr * F_rear;

    %% 2 滑转率损失

    
    % 只保留联盟中的驱动轮滑转率
    slip_active = abs(slip_s);

    % 防止空集导致 max([]) 问题
if sum(coalition) == 0

    lamdaN = 0;

else

    % 最大滑转率
    slip_max = max(slip_active);

    % 四次方强化惩罚
    lamdaN = slip_max^4;

end


    %% 3 附着利用率

    lambda_term = 0;

    for i = 1:4

        if coalition(i) == 1

            denom = uF_s(i);

            if abs(denom) > 1e-6

                lambda_i = Fx_s(i) / denom;

                % 平方强化
                lambda_term = ...
                    lambda_term + lambda_i^2;

            end

        end

    end

    %% 4 横摆力矩

    Mz = ...
        (-Fx_s(1) + Fx_s(2)) * bf + ...
        (-Fx_s(3) + Fx_s(4)) * br;

    %Mz = 

    %% 5 价值函数

    V_all(k) = ...
        traction_term ...
        - w1 * lamdaN ...
        + w2 * lambda_term ...
        - w3 * (Mz - Mz_ref)^2;

    Traction_all(k) = traction_term;
    lamdaN_all(k) = -w1 * lamdaN;
    lamda_all(k) = w2 * lambda_term;
    Mz_all(k) = - w3 * (Mz - Mz_ref)^2;

end

end

== matlab function tractor_mu2018/软土分配策略/MATLAB Function ==
  data: wheel_speeds_rpm input; selected_torques_n_m output; front_steer_angles_deg input; longitudinal_speed_mps input; applied_torques_n_m input; drive_torque_enabled input; baseline_torques_n_m input; wheel_torque_limits_n_m input; control_kappa output; filtered_kappa output; kappa_valid output; adaptive_targets output; cbf_torque_upper_bounds output; cbf_active output; nominal_torques_n_m output; soft_diag output
function [selected_torques_n_m, control_kappa, filtered_kappa, kappa_valid, adaptive_targets, cbf_torque_upper_bounds, cbf_active, nominal_torques_n_m, soft_diag] = shiche_soft_soil_adaptive_allocation(wheel_speeds_rpm, front_steer_angles_deg, longitudinal_speed_mps, applied_torques_n_m, drive_torque_enabled, baseline_torques_n_m, wheel_torque_limits_n_m)
%SHICHE_SOFT_SOIL_ADAPTIVE_ALLOCATION Real-vehicle soft-soil clamp allocator.
%
% MATLAB Function block version for VCU code generation. All numeric states,
% constants, intermediate arrays, and outputs are single precision.
%
% Wheel vector order is fixed as a 4x1 column:
%   [L1, R1, L2, R2] = [left-front, right-front, left-rear, right-rear]
%
% This block assumes an upstream load-based/basic four-wheel torque allocator
% already exists. baseline_torques_n_m is used as the reproducible anchor
% allocation. This real-vehicle version intentionally avoids QP, matrix solves,
% and active-set enumeration: it applies slip-tracking torque correction and
% then clamps each wheel by the CBF safety upper bound.
%
% Inputs:
%   wheel_speeds_rpm        single, 4x1 wheel speeds in rpm, [L1 R1 L2 R2].
%   front_steer_angles_deg  single, [Steer_L1 Steer_R1] in deg, or one scalar.
%   longitudinal_speed_mps  single, vehicle longitudinal speed in m/s.
%   applied_torques_n_m     single, 4x1 actual or one-step delayed applied wheel
%                           torques in N*m, [L1 R1 L2 R2].
%   drive_torque_enabled    single flag, >0.5 enables adaptive update and CBF.
%   baseline_torques_n_m    single, 4x1 upstream basic allocation in N*m.
%   wheel_torque_limits_n_m single, 4x1 nonnegative wheel torque limits in N*m.
%
% Outputs are single. kappa_valid and cbf_active are 0/1 single flags. soft_diag
% has 26 entries:
%   1:6   front target, rear target, simplified allocator status, total torque
%         reduction by CBF clamp, baseline total torque, selected total torque
%   7:10  filtered slip derivatives
%   11:14 slip input gains
%   15:18 slip disturbance estimates
%   19:22 disturbance margins
%   23:26 wheel surface speeds

persistent has_filtered filtered_state filtered_dot_state disturbance_state

if isempty(has_filtered)
    has_filtered = zeros(4, 1, 'single');
    filtered_state = zeros(4, 1, 'single');
    filtered_dot_state = zeros(4, 1, 'single');
    disturbance_state = zeros(4, 1, 'single');
end

dt = single(0.02);
wheel_speeds = column4_local(wheel_speeds_rpm);
front_steers = front_steer_pair_local(front_steer_angles_deg);
control_vx = single(longitudinal_speed_mps);
applied_torques = column4_local(applied_torques_n_m);
base_torques = column4_local(baseline_torques_n_m);
wheel_limits = column4_local(wheel_torque_limits_n_m);
drive_enabled = single(drive_torque_enabled) > single(0.5);

for index = 1:4
    wheel_limits(index) = max(single(0.0), wheel_limits(index));
    base_torques(index) = clamp_local(base_torques(index), single(0.0), wheel_limits(index));
end

[control_kappa, filtered_kappa, kappa_valid, dot_kappa, rolling_speeds, wheel_omegas, surface_speeds, has_filtered, filtered_state, filtered_dot_state] = ...
    update_slip_local(wheel_speeds, front_steers, control_vx, dt, has_filtered, filtered_state, filtered_dot_state);

front_target_base = single(0.078);
rear_target_base = single(0.128);
adaptive_targets = zeros(4, 1, 'single');
adaptive_targets(1) = front_target_base;
adaptive_targets(2) = front_target_base;
adaptive_targets(3) = rear_target_base;
adaptive_targets(4) = rear_target_base;

input_gains = input_gains_local(kappa_valid, rolling_speeds, wheel_omegas);
[disturbance_state, disturbance_margins] = update_disturbance_local(kappa_valid, dot_kappa, input_gains, applied_torques, dt, disturbance_state);

front_error = axle_slip_error_local(filtered_kappa, kappa_valid, adaptive_targets(1), 1);
rear_error = axle_slip_error_local(filtered_kappa, kappa_valid, adaptive_targets(3), 2);

nominal_torques_n_m = zeros(4, 1, 'single');
cbf_torque_upper_bounds = zeros(4, 1, 'single');
cbf_active = zeros(4, 1, 'single');
for index = 1:4
    gain = input_gains(index);
    if drive_enabled && kappa_valid(index) > single(0.5) && isfinite(gain)
        if index <= 2
            axle_error = front_error;
        else
            axle_error = rear_error;
        end
        torque_delta = clamp_local(-single(20500.0) * axle_error, -single(2600.0), single(2600.0));
        nominal = base_torques(index) + torque_delta;
    else
        nominal = base_torques(index);
    end
    nominal_torques_n_m(index) = clamp_local(nominal, single(0.0), wheel_limits(index));

    if drive_enabled && kappa_valid(index) > single(0.5) && isfinite(gain)
        upper = (single(15.0) * (single(0.25) - filtered_kappa(index)) - disturbance_state(index) - disturbance_margins(index)) / gain;
        if ~isfinite(upper)
            upper = wheel_limits(index);
        end
        upper = clamp_local(upper, single(0.0), wheel_limits(index));
    else
        upper = wheel_limits(index);
    end
    cbf_torque_upper_bounds(index) = upper;
    if upper < base_torques(index) - single(1.0e-6)
        cbf_active(index) = single(1.0);
    end
end

selected_torques_n_m = zeros(4, 1, 'single');
for index = 1:4
    selected_torques_n_m(index) = clamp_local(nominal_torques_n_m(index), single(0.0), cbf_torque_upper_bounds(index));
end

allocator_status = single(1.0);
total_torque_reduction = sum(nominal_torques_n_m - selected_torques_n_m);
baseline_total_torque = sum(base_torques);
selected_total_torque = sum(selected_torques_n_m);

soft_diag = zeros(26, 1, 'single');
soft_diag(1) = front_target_base;
soft_diag(2) = rear_target_base;
soft_diag(3) = allocator_status;
soft_diag(4) = total_torque_reduction;
soft_diag(5) = baseline_total_torque;
soft_diag(6) = selected_total_torque;
for index = 1:4
    soft_diag(6 + index) = dot_kappa(index);
    soft_diag(10 + index) = input_gains(index);
    soft_diag(14 + index) = disturbance_state(index);
    soft_diag(18 + index) = disturbance_margins(index);
    soft_diag(22 + index) = surface_speeds(index);
end
end

function [raw_kappa, filtered_kappa, valid, dot_kappa, rolling_speeds, omegas, surface_speeds, has_filtered_out, filtered_state_out, filtered_dot_out] = update_slip_local(wheel_speeds, front_steers, vx_mps, dt, has_filtered_in, filtered_state_in, filtered_dot_in)
rpm_to_rad = single(2.0) * single(pi) / single(60.0);
radii = zeros(4, 1, 'single');
radii(1) = single(0.834);
radii(2) = single(0.834);
radii(3) = single(0.94);
radii(4) = single(0.94);
speed_abs = abs(single(vx_mps));
steer_l = front_steers(1) * single(pi) / single(180.0);
steer_r = front_steers(2) * single(pi) / single(180.0);
rolling_speeds = zeros(4, 1, 'single');
rolling_speeds(1) = abs(speed_abs * cos(steer_l));
rolling_speeds(2) = abs(speed_abs * cos(steer_r));
rolling_speeds(3) = speed_abs;
rolling_speeds(4) = speed_abs;
omegas = abs(single(wheel_speeds)) * rpm_to_rad;
surface_speeds = radii .* omegas;

raw_kappa = zeros(4, 1, 'single');
filtered_kappa = zeros(4, 1, 'single');
dot_kappa = zeros(4, 1, 'single');
valid = zeros(4, 1, 'single');
has_filtered_out = has_filtered_in;
filtered_state_out = filtered_state_in;
filtered_dot_out = filtered_dot_in;
for index = 1:4
    raw_kappa(index) = single(NaN);
    filtered_kappa(index) = single(NaN);
end

alpha_kappa = first_order_alpha_local(dt, single(0.04));
alpha_dot = first_order_alpha_local(dt, single(0.08));
for index = 1:4
    is_valid = speed_abs >= single(0.08) && surface_speeds(index) >= single(0.20) && isfinite(rolling_speeds(index)) && isfinite(surface_speeds(index));
    if is_valid
        valid(index) = single(1.0);
        raw_value = single(1.0) - rolling_speeds(index) / surface_speeds(index);
        raw_kappa(index) = clamp_local(raw_value, -single(1.0), single(1.0));
        if has_filtered_in(index) <= single(0.5) || ~isfinite(filtered_state_in(index))
            filtered_value = raw_kappa(index);
            raw_dot = single(0.0);
        else
            previous = filtered_state_in(index);
            filtered_value = previous + alpha_kappa * (raw_kappa(index) - previous);
            raw_dot = (filtered_value - previous) / dt;
        end
        filtered_dot_out(index) = filtered_dot_in(index) + alpha_dot * (raw_dot - filtered_dot_in(index));
        filtered_state_out(index) = filtered_value;
        has_filtered_out(index) = single(1.0);
        filtered_kappa(index) = filtered_value;
        dot_kappa(index) = filtered_dot_out(index);
    else
        if has_filtered_in(index) > single(0.5)
            raw_kappa(index) = filtered_state_in(index);
            filtered_kappa(index) = filtered_state_in(index);
        end
        filtered_dot_out(index) = single(0.0);
        dot_kappa(index) = single(0.0);
    end
end
end

function front_steers = front_steer_pair_local(front_steer_angles_deg)
% Accept [Steer_L1, Steer_R1] or one equivalent front-axle steer angle.
steer_input = single(front_steer_angles_deg);
front_steers = zeros(2, 1, 'single');
if numel(steer_input) >= 2
    front_steers(1) = steer_input(1);
    front_steers(2) = steer_input(2);
else
    front_steers(1) = steer_input(1);
    front_steers(2) = steer_input(1);
end
end

function gains = input_gains_local(valid, rolling_speeds, omegas)
radii = zeros(4, 1, 'single');
radii(1) = single(0.834);
radii(2) = single(0.834);
radii(3) = single(0.94);
radii(4) = single(0.94);
inertias = zeros(4, 1, 'single');
inertias(1) = single(450.0);
inertias(2) = single(450.0);
inertias(3) = single(650.0);
inertias(4) = single(650.0);
gains = zeros(4, 1, 'single');
for index = 1:4
    gains(index) = single(NaN);
end
for index = 1:4
    if valid(index) > single(0.5) && omegas(index) > single(0.0)
        gain = rolling_speeds(index) / (inertias(index) * radii(index) * omegas(index) * omegas(index));
        if gain >= single(1.0e-8)
            gains(index) = gain;
        end
    end
end
end

function [disturbance_out, margins] = update_disturbance_local(valid, dot_kappa, input_gains, applied_torques, dt, disturbance_in)
disturbance_out = disturbance_in;
margins = zeros(4, 1, 'single');
alpha_disturbance = first_order_alpha_local(dt, single(0.15));
for index = 1:4
    gain = input_gains(index);
    if valid(index) > single(0.5) && isfinite(gain)
        raw_estimate = dot_kappa(index) - gain * applied_torques(index);
        disturbance_out(index) = disturbance_in(index) + alpha_disturbance * (raw_estimate - disturbance_in(index));
        residual = raw_estimate - disturbance_out(index);
    else
        residual = single(0.0);
    end
    margins(index) = clamp_local(single(0.05) + single(0.05) * abs(residual), single(0.05), single(5.0));
end
end

function error = axle_slip_error_local(filtered_kappa, valid, target, axle_id)
total = single(0.0);
count = single(0.0);
if axle_id == 1
    start_index = 1;
    end_index = 2;
else
    start_index = 3;
    end_index = 4;
end
for index = start_index:end_index
    if valid(index) > single(0.5) && isfinite(filtered_kappa(index))
        total = total + filtered_kappa(index);
        count = count + single(1.0);
    end
end
if count > single(0.0)
    error = total / count - target;
else
    error = single(0.0);
end
end

function alpha = first_order_alpha_local(dt, time_constant_s)
if dt <= single(0.0) || time_constant_s <= single(0.0)
    alpha = single(1.0);
else
    alpha = dt / (time_constant_s + dt);
end
end

function value = clamp_local(value_in, lower, upper)
value = min(max(single(value_in), single(lower)), single(upper));
end

function output = column4_local(values)
input_values = single(values);
output = zeros(4, 1, 'single');
for index = 1:4
    output(index) = input_values(index);
end
end

== stateflow chart tractor_mu2018/总驱动力矩制定/负载工况_极限防抖 ==
  state Normal
    entry:
    T_hold = 0;
    during:
    T0_out = T0;
  state Limit_detect
    during:
    T0_out = T0;
  state Limit_hold
    entry:
    T_hold = T0;
    during:
    T_hold = T_hold + 0.02*(T0 - T_hold);
    T_hold = min(max(T_hold,2000),60000);
    T0_out = T_hold;
  (default) -> Normal
  Limit_detect -> Normal [order 1] : [(throttle < 0.7) || (load_rate < 0.9) || (abs(ax) > 0.1)]
  Normal -> Limit_detect : [(throttle > 0.8) && (load_rate > 0.9) && (abs(ax) < 0.1) ]
  Limit_hold -> Normal : [ (load_rate < 0.85) && (abs(ax) > 0.12)]
  Limit_detect -> Limit_hold [order 2] : [after(0.5,sec)]
  data: throttle input; ax input; Tmax input; load_rate input; T0 input; T0_out output; T_hold local; timer_start local

== matlab function tractor_mu2018/PID_Controller//直线循迹/MATLAB Function ==
  data: u input; y output
function y = lowpass_filter(u)
persistent prev_x prev_y;
if isempty(prev_x), prev_x = 0; end
if isempty(prev_y), prev_y = 0; end

% 差分方程: y(n) = 0.2452*u(n) + 0.2452*u(n-1) + 0.5095*y(n-1)
y = 0.2452*u + 0.2452*prev_x + 0.5095*prev_y;

% 更新状态
prev_x = double(u);
prev_y = double(y);
end
